simulink model "advanced_active_clamping"  (R2023b)
settings: Solver=ode1be  StartTime=0.0  StopTime=simlength  FixedStep=tc  RelTol=1e-3
values from neighbouring files (symbols this model uses):
  Rgate = 2.5    [init_model.m]
  Rgate_internal = 4    [init_model.m]
  t0_dpt = 5e-6    (= 5e-06)    [init_model.m]
  t1_dpt = t0_dpt + delta_time_first_pulse    (= 0.000105)    [init_model.m]
  t2_dpt = t1_dpt + deadtime    (= 0.000108)    [init_model.m]
  t3_dpt = t2_dpt + delta_time_discharge    (= 0.000128)    [init_model.m]
  t4_dpt = t3_dpt + deadtime    (= 0.000131)    [init_model.m]
  t5_dpt = t4_dpt + delta_time_second_pulse    (= 0.000166)    [init_model.m]
  t6_dpt = t5_dpt + deadtime    (= 0.000169)    [init_model.m]
  Vdc = 1400    [init_model.m]
  Vgate_h = 15    [init_model.m]
  Vgate_l = -7    [init_model.m]
libraries: fl_lib x55, nesl_utility x11, ee_lib x10, simulink x4
(part 1 of 3)
settings Model: SimulationMode=accelerator  Creator=ltnbda  LastModifiedBy=ltnbda

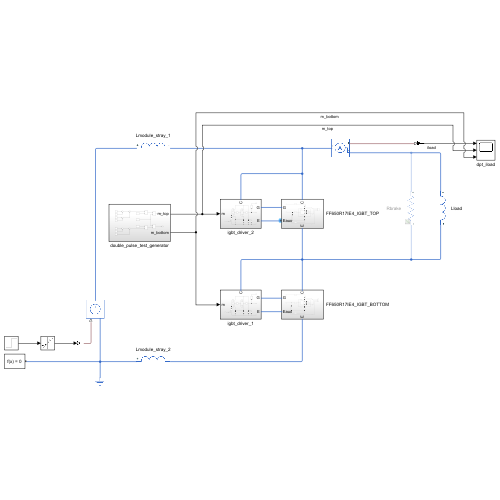
[thumbnail: Simulink's stored preview of the top-level diagram]
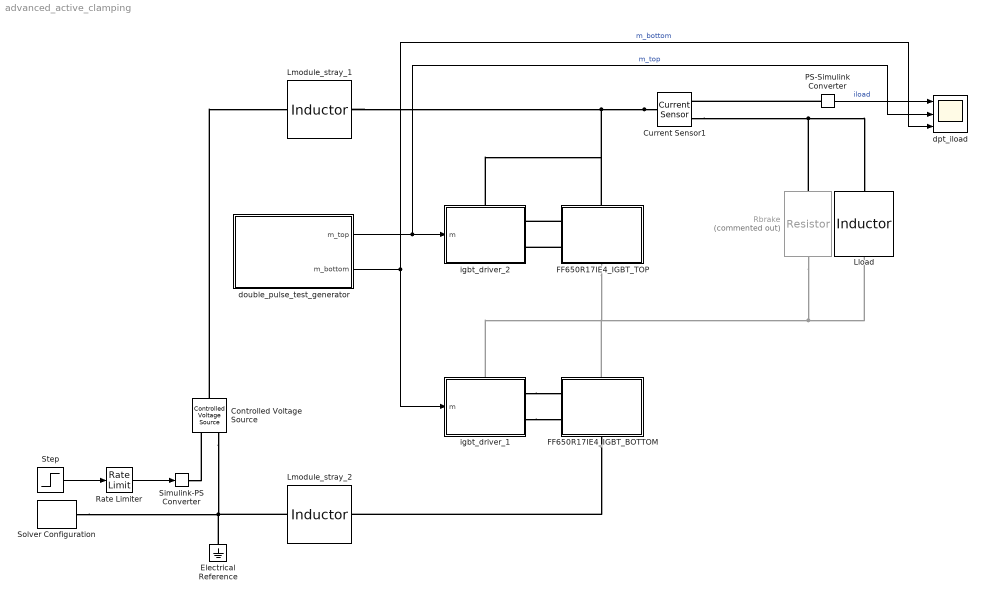
== system advanced_active_clamping ==
  Controlled Voltage Source : fl_lib/Electrical/Electrical Sources/Controlled Voltage Source
  Current Sensor1 : fl_lib/Electrical/Electrical Sensors/Current Sensor
  Electrical Reference : fl_lib/Electrical/Electrical Elements/Electrical Reference
  FF650R17IE4_IGBT_BOTTOM : Subsystem
      settings: PortSchema="{\"entries\":[{\"content\":{\"sides\":[{\"content\":{\"connectorIds\":[\"LConn1\",\"LConn2\"]},\"type\":\"ConnectorPlacement.EquallySpacedRectSide\",\"uuid\":\"ff7886c7-4f8e-447f-95ba-85dce919debf\"},{\"content\":{\"side\":\"RIGHT\"},\"type\":\"ConnectorPlacement.EquallySpacedRectSide\",\"uuid\":\"5b5ddf05-2751-4064-9c00-5bb01a041ae0\"},{\"content\":{\"connectorIds\":[\"LConn3\"],\"side\":\"TOP\"},\"type\":\"ConnectorPlacement.EquallySpacedRectSide\",\"uuid\":\"273e317c-7515-4411-a6b6-783120e9a5d2\"},{\"content\":{\"connectorIds\":[\"RConn1\"],\"side\":\"BOTTOM\"},\"type\":\"ConnectorPlacement.EquallySpacedRectSide\",\"uuid\":\"19a3252d-8455-4daa-8248-ea8f9abc4bb8\"}]},\"type\":\"ConnectorPlacement.EquallySpacedConnector\",\"uuid\":\"2d9de646-1f96-414a-bd08-ff96b52427d0\"}],\"packageUris\":[\"http://schema.mathworks.com/mf0/Connector/R2020b\"],\"version\":\"1.0\"}"
  FF650R17IE4_IGBT_TOP : Subsystem
      settings: PortSchema="{\"entries\":[{\"content\":{\"sides\":[{\"content\":{\"connectorIds\":[\"LConn1\",\"LConn2\"]},\"type\":\"ConnectorPlacement.EquallySpacedRectSide\",\"uuid\":\"ff7886c7-4f8e-447f-95ba-85dce919debf\"},{\"content\":{\"side\":\"RIGHT\"},\"type\":\"ConnectorPlacement.EquallySpacedRectSide\",\"uuid\":\"5b5ddf05-2751-4064-9c00-5bb01a041ae0\"},{\"content\":{\"connectorIds\":[\"LConn3\"],\"side\":\"TOP\"},\"type\":\"ConnectorPlacement.EquallySpacedRectSide\",\"uuid\":\"273e317c-7515-4411-a6b6-783120e9a5d2\"},{\"content\":{\"connectorIds\":[\"RConn1\"],\"side\":\"BOTTOM\"},\"type\":\"ConnectorPlacement.EquallySpacedRectSide\",\"uuid\":\"19a3252d-8455-4daa-8248-ea8f9abc4bb8\"}]},\"type\":\"ConnectorPlacement.EquallySpacedConnector\",\"uuid\":\"2d9de646-1f96-414a-bd08-ff96b52427d0\"}],\"packageUris\":[\"http://schema.mathworks.com/mf0/Connector/R2020b\"],\"version\":\"1.0\"}"
  Lload : fl_lib/Electrical/Electrical Elements/Inductor  l=250e-6 H  r=0 Ohm  g=1e-9 1/Ohm  i_specify=on  i_priority=High  i=0 A  i_nominal_specify=off  i_nominal_unit=A  i_nominal_value=1  v_specify=off  v_priority=None  v=0 V  v_nominal_specify=off  v_nominal_unit=V  v_nominal_value=1  i_L_specify=off  i_L_priority=High  i_L=0 A  i_L_nominal_specify=off  i_L_nominal_unit=A  i_L_nominal_value=1
  Lmodule_stray_1 : fl_lib/Electrical/Electrical Elements/Inductor  l=10e-9 H  r=0 Ohm  g=1e-9 1/Ohm  i_specify=on  i_priority=High  i=0 A  i_nominal_specify=off  i_nominal_unit=A  i_nominal_value=1  v_specify=off  v_priority=None  v=0 V  v_nominal_specify=off  v_nominal_unit=V  v_nominal_value=1  i_L_specify=off  i_L_priority=High  i_L=0 A  i_L_nominal_specify=off  i_L_nominal_unit=A  i_L_nominal_value=1
  Lmodule_stray_2 : fl_lib/Electrical/Electrical Elements/Inductor  l=10e-9 H  r=0 Ohm  g=1e-9 1/Ohm  i_specify=on  i_priority=High  i=0 A  i_nominal_specify=off  i_nominal_unit=A  i_nominal_value=1  v_specify=off  v_priority=None  v=0 V  v_nominal_specify=off  v_nominal_unit=V  v_nominal_value=1  i_L_specify=off  i_L_priority=High  i_L=0 A  i_L_nominal_specify=off  i_L_nominal_unit=A  i_L_nominal_value=1
  PS-Simulink Converter : nesl_utility/PS-Simulink Converter  PhysicalDomain=network_engine_domain  SubClassName=ps_output  LeftPortType=input  RightPortType=output  PseudoPeriodic=off  Frequencies=[]  VectorFormat=1-D array  Unit=A  AffineConversion=off
  Rate Limiter : RateLimiter  RisingSlewLimit=Vdc/t0_dpt  FallingSlewLimit=-Vdc/t0_dpt  SampleTimeMode=inherited
  Rbrake : fl_lib/Electrical/Electrical Elements/Resistor  Commented=on  R=2.5 Ohm  i_specify=off  i_priority=None  i=0 A  i_nominal_specify=off  i_nominal_unit=A  i_nominal_value=1  v_specify=off  v_priority=None  v=0 V  v_nominal_specify=off  v_nominal_unit=V  v_nominal_value=1
  Simulink-PS Converter : nesl_utility/Simulink-PS Converter  PhysicalDomain=network_engine_domain  SubClassName=ps_input  LeftPortType=input  RightPortType=output  PseudoPeriodic=off  Frequencies=[]  NoiseDistribution=none  NoiseParameters=[]  Unit=V  AffineConversion=off  FilteringAndDerivatives=provide  SimscapeFilterOrder=1  InputFilterTimeConstant=0.001  UdotUserProvided=0
  Solver Configuration : nesl_utility/Solver Configuration  PhysicalDomain=network_engine_domain  SubClassName=solver  LeftPortType=input  RightPortType=generic  Tones=[]  Harmonics=[]  SimulateNoise=off  Profile=off  UseLocalSampling=off  EnableSwitchedLinearOptims=on  FrequencyDomain=off  UseCCode=off  RelTol=0.001  AbsTol=0.001  MinStep=1e-09  ToWorkspace=off  RevertToSquareIcSolve=off  NumHomotopyIterations=100  PhasorMode=off  PhasorModeNumHarmonics=1  ConsistencySolver=NEWTON_XTOL_AFTER_FTOL  IndexReductionMethod=DerivativeReplacement  DoDC=off  ResidualTolerance=1e-09  ConsistencyTolSource=GLOBAL  ConsistencyAbsTol=0.001  ConsistencyRelTol=0.001  ConsistencyTolFactor=0.001  UseLocalSolver=on  LocalSolverChoice=NE_BACKWARD_EULER_ADVANCER  ResolveIndetEquations=on  FunctionEvalNumThread=1  LocalSolverSampleTime=tc  DoFixedCost=on  MaxNonlinIter=3  MaxModeIter=2  ComputeImpulses=off  ImpulseIterations=2  LinearAlgebra=auto  LinearAlgebraNumThread=0  EquationFormulation=NE_TIME_EF  DelaysMemoryBudget=1024  AutomaticFiltering=on  FilteringTimeConstant=0.001  PartitionStorageMethod=AS_NEEDED  PartitionMemoryBudget=1024  PartitionMethod=ROBUST  MultibodyUseLocalSolver=off  MultibodyLocalSolverChoice=ODE1  MultibodyLocalSolverSampleTime=0.001
  Step : Step  Time=t0_dpt/2  After=Vdc  SampleTime=0
  double_pulse_test_generator : Subsystem
  dpt_iload : Scope  NumInputPorts=3
  igbt_driver_1 : Subsystem
      settings: PortSchema="{\"entries\":[{\"content\":{\"sides\":[{\"content\":{\"connectorIds\":[\"In1\"]},\"type\":\"ConnectorPlacement.EquallySpacedRectSide\",\"uuid\":\"b5509b55-d3cc-4efd-9891-ed827e6493bc\"},{\"content\":{\"connectorIds\":[\"RConn1\",\"RConn2\"],\"side\":\"RIGHT\"},\"type\":\"ConnectorPlacement.EquallySpacedRectSide\",\"uuid\":\"dc61ae1f-7170-4116-bac1-734370f471cc\"},{\"content\":{\"connectorIds\":[\"LConn1\"],\"side\":\"TOP\"},\"type\":\"ConnectorPlacement.EquallySpacedRectSide\",\"uuid\":\"cf9a77ed-ea6e-4e11-a579-61eb3ec7e471\"},{\"content\":{\"side\":\"BOTTOM\"},\"type\":\"ConnectorPlacement.EquallySpacedRectSide\",\"uuid\":\"ce6ad74e-4413-41a4-ad14-2bad8f537036\"}]},\"type\":\"ConnectorPlacement.EquallySpacedConnector\",\"uuid\":\"97660843-38c1-4e0d-9e7b-61942c4360f8\"}],\"packageUris\":[\"http://schema.mathworks.com/mf0/Connector/R2020b\"],\"version\":\"1.0\"}"
  igbt_driver_2 : Subsystem
      settings: PortSchema="{\"entries\":[{\"content\":{\"sides\":[{\"content\":{\"connectorIds\":[\"In1\"]},\"type\":\"ConnectorPlacement.EquallySpacedRectSide\",\"uuid\":\"b5509b55-d3cc-4efd-9891-ed827e6493bc\"},{\"content\":{\"connectorIds\":[\"RConn1\",\"RConn2\"],\"side\":\"RIGHT\"},\"type\":\"ConnectorPlacement.EquallySpacedRectSide\",\"uuid\":\"dc61ae1f-7170-4116-bac1-734370f471cc\"},{\"content\":{\"connectorIds\":[\"LConn1\"],\"side\":\"TOP\"},\"type\":\"ConnectorPlacement.EquallySpacedRectSide\",\"uuid\":\"cf9a77ed-ea6e-4e11-a579-61eb3ec7e471\"},{\"content\":{\"side\":\"BOTTOM\"},\"type\":\"ConnectorPlacement.EquallySpacedRectSide\",\"uuid\":\"ce6ad74e-4413-41a4-ad14-2bad8f537036\"}]},\"type\":\"ConnectorPlacement.EquallySpacedConnector\",\"uuid\":\"97660843-38c1-4e0d-9e7b-61942c4360f8\"}],\"packageUris\":[\"http://schema.mathworks.com/mf0/Connector/R2020b\"],\"version\":\"1.0\"}"
  wires:
  Step/1 -> Rate Limiter/1
  double_pulse_test_generator/2(m_bottom) -> igbt_driver_1/1(m), dpt_iload/3  "m_bottom"
  double_pulse_test_generator/1(m_top) -> igbt_driver_2/1(m), dpt_iload/2  "m_top"
  PS-Simulink Converter/1 -> dpt_iload/1  "iload"
  Rate Limiter/1 -> Simulink-PS Converter/1
  connections:
  Current Sensor1/LConn1 -- igbt_driver_2/LConn1 -- FF650R17IE4_IGBT_TOP/LConn3 -- Lmodule_stray_1/RConn1
  Simulink-PS Converter/RConn1 -- Controlled Voltage Source/RConn1
  FF650R17IE4_IGBT_BOTTOM/RConn1 -- Lmodule_stray_2/RConn1
  Rbrake/RConn1 -- igbt_driver_1/LConn1 -- FF650R17IE4_IGBT_BOTTOM/LConn3 -- FF650R17IE4_IGBT_TOP/RConn1 -- Lload/RConn1
  igbt_driver_1/RConn1 -- FF650R17IE4_IGBT_BOTTOM/LConn1
  FF650R17IE4_IGBT_TOP/LConn1 -- igbt_driver_2/RConn1
  Current Sensor1/RConn2 -- Rbrake/LConn1 -- Lload/LConn1
  PS-Simulink Converter/LConn1 -- Current Sensor1/RConn1
  Controlled Voltage Source/LConn1 -- Lmodule_stray_1/LConn1
  Lmodule_stray_2/LConn1 -- Electrical Reference/LConn1 -- Controlled Voltage Source/RConn2 -- Solver Configuration/RConn1
  igbt_driver_1/RConn2 -- FF650R17IE4_IGBT_BOTTOM/LConn2
  FF650R17IE4_IGBT_TOP/LConn2 -- igbt_driver_2/RConn2

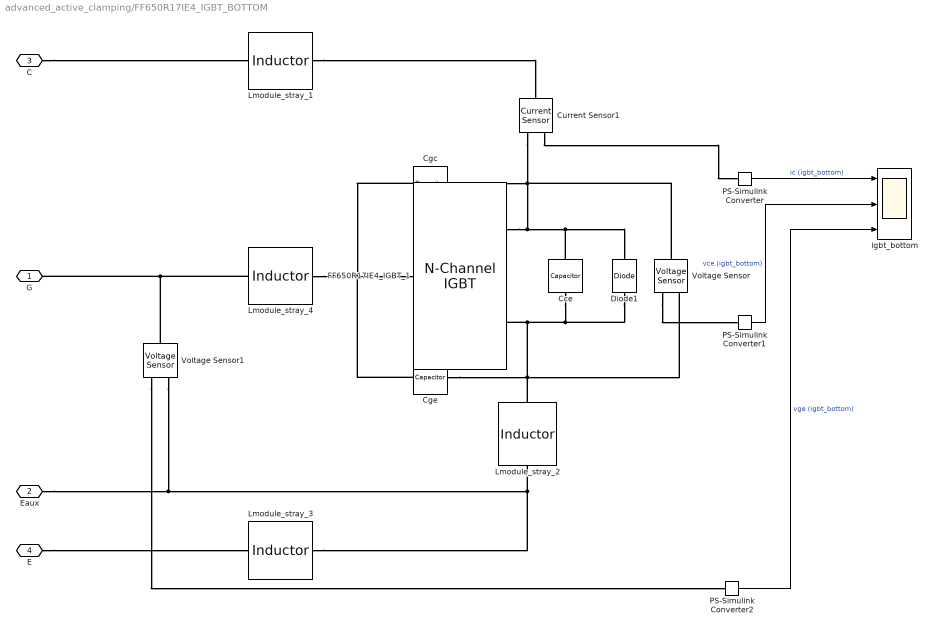
== system advanced_active_clamping/FF650R17IE4_IGBT_BOTTOM ==
  Cce : fl_lib/Electrical/Electrical Elements/Capacitor  c=Cce F  r=RCce Ohm  g=0 1/Ohm  i_specify=off  i_priority=None  i=0 A  i_nominal_specify=off  i_nominal_unit=A  i_nominal_value=1  v_specify=off  v_priority=None  v=0 V  v_nominal_specify=off  v_nominal_unit=V  v_nominal_value=1  vc_specify=off  vc_priority=High  vc=0 V  vc_nominal_specify=off  vc_nominal_unit=V  vc_nominal_value=1
  Cgc : fl_lib/Electrical/Electrical Elements/Capacitor  c=Cgc F  r=RCgc Ohm  g=0 1/Ohm  i_specify=off  i_priority=None  i=0 A  i_nominal_specify=off  i_nominal_unit=A  i_nominal_value=1  v_specify=off  v_priority=None  v=0 V  v_nominal_specify=off  v_nominal_unit=V  v_nominal_value=1  vc_specify=off  vc_priority=High  vc=0 V  vc_nominal_specify=off  vc_nominal_unit=V  vc_nominal_value=1
  Cge : fl_lib/Electrical/Electrical Elements/Capacitor  c=Cge F  r=RCge Ohm  g=0 1/Ohm  i_specify=off  i_priority=None  i=0 A  i_nominal_specify=off  i_nominal_unit=A  i_nominal_value=1  v_specify=off  v_priority=None  v=0 V  v_nominal_specify=off  v_nominal_unit=V  v_nominal_value=1  vc_specify=off  vc_priority=High  vc=0 V  vc_nominal_specify=off  vc_nominal_unit=V  vc_nominal_value=1
  Current Sensor1 : fl_lib/Electrical/Electrical Sensors/Current Sensor
  Diode1 : fl_lib/Electrical/Electrical Elements/Diode  Vf=2 V  Ron=0.3 Ohm  Goff=1e-8 1/Ohm  i_specify=off  i_priority=None  i=0 A  i_nominal_specify=off  i_nominal_unit=A  i_nominal_value=1  v_specify=off  v_priority=None  v=0 V  v_nominal_specify=off  v_nominal_unit=V  v_nominal_value=1
  FF650R17IE4_IGBT_1 : ee_lib/Semiconductors & Converters/N-Channel IGBT  model_type=ee.enum.igbt.parameterization.equation  Ices=5 mA  Vces=1700 V  Vth=5.8 V  Vce_sat=2.35 V  Ice_sat=650 A  Vge_sat=15 V  Tmeas=125 degC  Vge_vec=[-1, 0, 2, 3, 5, 6, 7, 8, 10, 12, 15, 18, 20] V  Vce_vec=[0, .25, .5, .75, 1, 1.26, 1.51, 1.76, 2.01, 2.26, 2.51, 2.76, 3.01, 3.27, 3.52, 3.77, 4.02, 4.27, 4.52, 4.77] V  T_vec=[25, 125] degC  Ic_mat=[0, 0, 0, 0, 0, 0, 0, 0, 0, 0, 0, 0, 0, 0, 0, 0, 0, 0, 0, 0; 0, 0, 0, 0, 0, 0, 0, 0, 0, 0, 0, 0, 0, 0, 0, 0, 0, 0, 0, 0; 0, 0, 0, 0, 0, 0, 0, 0, 0, 0, 0, 0, 0, 0, 0, 0, 0, 0, 0, 0; 0, 0, 0, 0, 0, 0, 0, 0, 0, 0, 0, 0, 0, 0, 0, 0, 0, 0, 0, 0; 0, 0, 0, 0, 0, 0, 0, 0, 0, 0, 0, 0, 0, 0, 0, 0, 0, 0, 0, 0; 0, 0, 0, .81, 3.13, 4.97, 6.03, 6.53, 6.84, 7.01, 7.19, 7.32, 7.44, 7.55, 7.67, 7.78, 7.89, 8, 8.07, 8.07; 0, 0, 0, 1.07, 5.5, 12.93, 22.09, 29.14, 35.27, 38.97, 41.37, 43.08, 44.52, 45.45, 46.28, 46.85, 47.41, 47.76, 48.06, 48.36; 0, 0, 0, 1.1, 6.99, 16.51, 28.38, 41.53, 55.76, 69.08, 80.5, 89.56, 96.13, 101.45, 105.15, 107.99, 110.09, 111.87, 113.54, 114.95; 0, 0, 0, 1.36, 6.26, 17.43, 33.6, 50.43, 71.75, 93.61, 114.64, 134.42, 151.44, 164.25, 177.06, 189.88, 202.69, 215.51, 228.32, 241.14; 0, 0, 0, 1.42, 6.4, 18.7, 36.19, 55.23, 79.71, 106.22, 131.28, 156.62, 182.79, 208.97, 235.15, 261.32, 287.5, 313.67, 339.85, 366.02; 0, 0, 0, 1.45, 6.81, 20.01, 39.61, 60.63, 88.74, 117.7, 147.16, 191.87, 237.14, 282.42, 327.69, 372.96, 418.23, 463.5, 508.77, 554.04; 0, 0, 0, 1.49, 6.97, 20.55, 41.34, 64.15, 94.91, 126.1, 170.16, 233.77, 297.38, 360.98, 424.59, 488.19, 551.8, 615.4, 679.01, 742.62; 0, 0, 0, 1.5, 7.5, 20.96, 42.17, 66.19, 98.34, 131.14, 187.84, 263.46, 339.09, 414.72, 490.34, 565.97, 641.6, 717.22, 792.85, 868.48] A  Ic_mat_3D=zeros(13, 20, 2) A  C_param=ee.enum.igbt.capacitanceParam.fixedciss  C_GE=23.7 nF  C_GC=2.7 nF  C_CE=0 nF  C_ies=54 nF  C_res=1.7 nF  C_oes=0 nF  C_GE_vec=[25, 31, 26.5, 24.9, 25, 24.9, 24.6, 24.7, 24.8] nF  C_GC_vec=[55, 9, 5.5, 3.1, 2.5, 2.1, 1.9, 1.8, 1.7] nF  C_Vge_vec=0 V  C_CE_vec=[5, 11, 6.5, 4.9, 3.5, 2.7, 2.1, 1.7, 1.4] nF  C_ies_vec=[80, 40, 32, 28, 27.5, 27, 26.5, 26.5, 26.5] nF  C_res_vec=[55, 9, 5.5, 3.1, 2.5, 2.1, 1.9, 1.8, 1.7] nF  C_oes_vec=[60, 20, 12, 8, 6, 4.8, 4, 3.5, 3.1] nF  C_Vce_vec=[0, 1, 2, 5, 10, 15, 20, 25, 30] V  charge_linearity_param=ee.enum.igbt.cgcLinearity.constant  C_OX=20 nF  V_C_OX=-5 V  TF=0 us  TT=0 us  ec=1  VAF=1 V  RC=0.001 Ohm  RE=0.001 Ohm  RG=2.3 Ohm  BF=50  T_param=ee.enum.igbt.temperatureParameterization.none  Ices_T2=100 mA  EG=1.11 eV  Vce_sat_T2=3 V  Tmeas2=125 degC  XTI=3  BEX=-1.5  RG_alpha=0 1/K  Tdevice=300 K  Tdevice_3D=25 degC  has_thermal_port=1  ig_specify=off  ig_priority=None  ig=0 A  ig_nominal_specify=off  ig_nominal_unit=A  ig_nominal_value=1  ic_specify=off  ic_priority=None  ic=0 A  ic_nominal_specify=off  ic_nominal_unit=A  ic_nominal_value=1  vge_specify=off  vge_priority=None  vge=0 V  vge_nominal_specify=off  vge_nominal_unit=V  vge_nominal_value=1  vce_specify=off  vce_priority=None  vce=0 V  vce_nominal_specify=off  vce_nominal_unit=V  vce_nominal_value=1  v_Cge_specify=off  v_Cge_priority=High  v_Cge=0 V  v_Cge_nominal_specify=off  v_Cge_nominal_unit=V  v_Cge_nominal_value=1  v_Cce_specify=off  v_Cce_priority=High  v_Cce=0 V  v_Cce_nominal_specify=off  v_Cce_nominal_unit=V  v_Cce_nominal_value=1  thermal_network_parameterization=ee.enum.thermalNetworkTopology.junctionCase  Rth=[0, 10] K/W  Rth_Cauer=[1, 3, 10] K/W  Rth_Foster=[4, 6] K/W  thermal_mass_parameterization=ee.enum.thermalNetwork.timeconstant  thermal_mass=[0, 1] J/K  thermal_mass_Cauer=[.1, .3, 1] J/K  thermal_mass_Foster=[1.5, 3] J/K  thermal_time_constant=[0, 10] s  thermal_time_constant_Cauer=[1, 3, 10] s  thermal_time_constant_Foster=[6, 18] s  thermal_mass_initial_temperatures=[25, 25] degC  thermal_mass_initial_temperatures_Cauer=[25, 25, 25] degC  Tvec_initial_Foster=[25, 25, 25, 25] degC  Ic_vec1=[0, 10, 50, 100, 200, 400, 600] A  Vce_vec1=[0, 1.1, 1.3, 1.45, 1.75, 2.25, 2.7] V  Rmiller=0.1 Ohm  Goff=1e-5 1/Ohm  t_on=0.07 us  t_rise=0.7 us  t_off=0.2 us  t_fall=0.5 us  v_meas=300 V  vStartTurnOn_specify=off  vStartTurnOn_priority=None  vStartTurnOn=1 V  tStartTurnOn_specify=off  tStartTurnOn_priority=None  tStartTurnOn=0 s  vStartTurnOff_specify=off  vStartTurnOff_priority=None  vStartTurnOff=0.5 V  tStartTurnOff_specify=off  tStartTurnOff_priority=None  tStartTurnOff=0 s  Tj_vec1=[298.15, 398.15] K  Vce_mat1=[0, 1.1, 1.3, 1.45, 1.75, 2.25, 2.7; 0, 1, 1.15, 1.35, 1.7, 2.35, 3] V  Tj_vec_loss=[298.15, 398.15] K  Ic_vec_loss=[0, 10, 50, 100, 200, 400, 600] A  E_turn_on_mat1=[0, .2, 1, 2, 4, 8, 15; 0, .3, 1.3, 2.5, 5, 11, 18] * 1e-3 J  E_turn_off_mat1=[0, .3, 1.5, 3, 6, 15, 25; 0, .7, 3.3, 6.5, 13, 25, 35] * 1e-3 J  iStartTurnOff_specify=off  iStartTurnOff_priority=None  iStartTurnOff=0 A  Tdevice_specify=off  Tdevice_priority=None
      settings: InternalSimscapePortConfiguration="{\"Bottom\":[],\"Left\":[{\"id\":\"G\",\"label\":\"\",\"type\":\"foundation.electrical.electrical\"}],\"Right\":[{\"id\":\"C\",\"label\":\"\",\"type\":\"foundation.electrical.electrical\"},{\"id\":\"E\",\"label\":\"\",\"type\":\"foundation.electrical.electrical\"}],\"Top\":[]}"
  Lmodule_stray_{1..4} (4 alike) : fl_lib/Electrical/Electrical Elements/Inductor  l=Lstray_module H  r=RLstray_module Ohm  g=1e-9 1/Ohm  i_specify=on  i_priority=High  i=0 A  i_nominal_specify=off  i_nominal_unit=A  i_nominal_value=1  v_specify=off  v_priority=None  v=0 V  v_nominal_specify=off  v_nominal_unit=V  v_nominal_value=1  i_L_specify=off  i_L_priority=High  i_L=0 A  i_L_nominal_specify=off  i_L_nominal_unit=A  i_L_nominal_value=1
  PS-Simulink Converter : nesl_utility/PS-Simulink Converter  PhysicalDomain=network_engine_domain  SubClassName=ps_output  LeftPortType=input  RightPortType=output  PseudoPeriodic=off  Frequencies=[]  VectorFormat=1-D array  Unit=A  AffineConversion=off
  PS-Simulink Converter1 : nesl_utility/PS-Simulink Converter  PhysicalDomain=network_engine_domain  SubClassName=ps_output  LeftPortType=input  RightPortType=output  PseudoPeriodic=off  Frequencies=[]  VectorFormat=1-D array  Unit=V  AffineConversion=off
  PS-Simulink Converter2 : nesl_utility/PS-Simulink Converter  PhysicalDomain=network_engine_domain  SubClassName=ps_output  LeftPortType=input  RightPortType=output  PseudoPeriodic=off  Frequencies=[]  VectorFormat=1-D array  Unit=V  AffineConversion=off
  Voltage Sensor : fl_lib/Electrical/Electrical Sensors/Voltage Sensor
  Voltage Sensor1 : fl_lib/Electrical/Electrical Sensors/Voltage Sensor
  igbt_bottom : Scope  NumInputPorts=3
  G : PMIOPort  Side=Left
  Eaux : PMIOPort  Port=2  Side=Left
  C : PMIOPort  Port=3  Side=Left
  E : PMIOPort  Port=4  Side=Right
  wires:
  PS-Simulink Converter2/1 -> igbt_bottom/3  "vge (igbt_bottom)"
  PS-Simulink Converter/1 -> igbt_bottom/1  "ic (igbt_bottom)"
  PS-Simulink Converter1/1 -> igbt_bottom/2  "vce (igbt_bottom)"
  connections:
  Lmodule_stray_2/RConn1 -- Voltage Sensor1/RConn2 -- Eaux/RConn1 -- Lmodule_stray_3/LConn1
  G/RConn1 -- Lmodule_stray_4/LConn1 -- Voltage Sensor1/LConn1
  FF650R17IE4_IGBT_1/RConn2 -- Cce/RConn1 -- Diode1/LConn1 -- Lmodule_stray_2/LConn1 -- Voltage Sensor/RConn2 -- Cge/RConn1
  E/RConn1 -- Lmodule_stray_3/RConn1
  C/RConn1 -- Lmodule_stray_1/LConn1
  Lmodule_stray_1/RConn1 -- Current Sensor1/LConn1
  FF650R17IE4_IGBT_1/LConn1 -- Lmodule_stray_4/RConn1 -- Cgc/LConn1 -- Cge/LConn1
  Voltage Sensor1/RConn1 -- PS-Simulink Converter2/LConn1
  Voltage Sensor/RConn1 -- PS-Simulink Converter1/LConn1
  Voltage Sensor/LConn1 -- Current Sensor1/RConn2 -- Cgc/RConn1 -- Diode1/RConn1 -- Cce/LConn1 -- FF650R17IE4_IGBT_1/RConn1
  Current Sensor1/RConn1 -- PS-Simulink Converter/LConn1

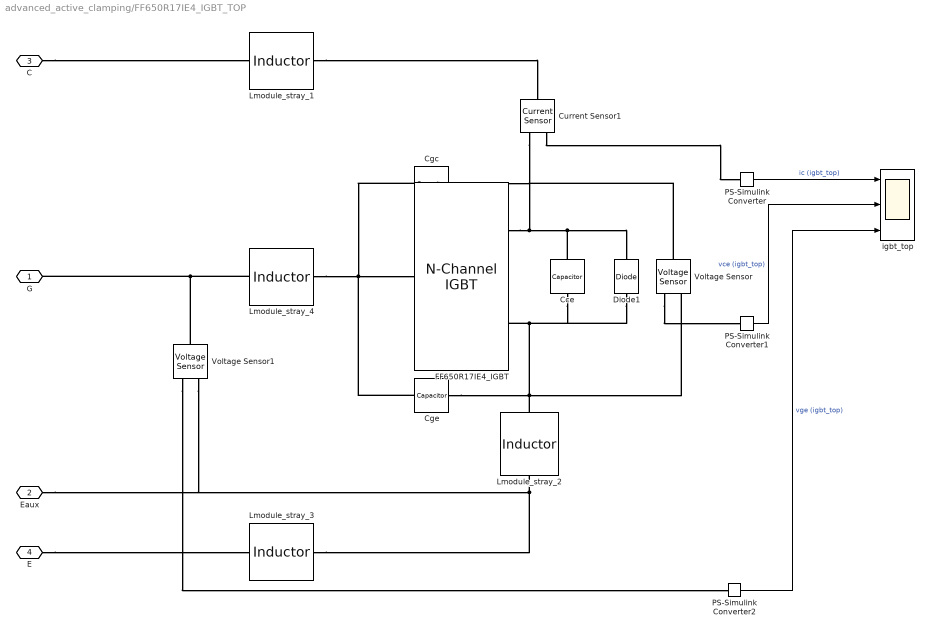
== system advanced_active_clamping/FF650R17IE4_IGBT_TOP ==
  Cce : fl_lib/Electrical/Electrical Elements/Capacitor  c=Cce F  r=RCce Ohm  g=0 1/Ohm  i_specify=off  i_priority=None  i=0 A  i_nominal_specify=off  i_nominal_unit=A  i_nominal_value=1  v_specify=off  v_priority=None  v=0 V  v_nominal_specify=off  v_nominal_unit=V  v_nominal_value=1  vc_specify=off  vc_priority=High  vc=0 V  vc_nominal_specify=off  vc_nominal_unit=V  vc_nominal_value=1
  Cgc : fl_lib/Electrical/Electrical Elements/Capacitor  c=Cgc F  r=RCgc Ohm  g=0 1/Ohm  i_specify=off  i_priority=None  i=0 A  i_nominal_specify=off  i_nominal_unit=A  i_nominal_value=1  v_specify=off  v_priority=None  v=0 V  v_nominal_specify=off  v_nominal_unit=V  v_nominal_value=1  vc_specify=off  vc_priority=High  vc=0 V  vc_nominal_specify=off  vc_nominal_unit=V  vc_nominal_value=1
  Cge : fl_lib/Electrical/Electrical Elements/Capacitor  c=Cge F  r=RCge Ohm  g=0 1/Ohm  i_specify=off  i_priority=None  i=0 A  i_nominal_specify=off  i_nominal_unit=A  i_nominal_value=1  v_specify=off  v_priority=None  v=0 V  v_nominal_specify=off  v_nominal_unit=V  v_nominal_value=1  vc_specify=off  vc_priority=High  vc=0 V  vc_nominal_specify=off  vc_nominal_unit=V  vc_nominal_value=1
  Current Sensor1 : fl_lib/Electrical/Electrical Sensors/Current Sensor
  Diode1 : fl_lib/Electrical/Electrical Elements/Diode  Vf=2 V  Ron=0.3 Ohm  Goff=1e-8 1/Ohm  i_specify=off  i_priority=None  i=0 A  i_nominal_specify=off  i_nominal_unit=A  i_nominal_value=1  v_specify=off  v_priority=None  v=0 V  v_nominal_specify=off  v_nominal_unit=V  v_nominal_value=1
  FF650R17IE4_IGBT : ee_lib/Semiconductors & Converters/N-Channel IGBT  model_type=ee.enum.igbt.parameterization.equation  Ices=5 mA  Vces=1700 V  Vth=5.8 V  Vce_sat=2.35 V  Ice_sat=650 A  Vge_sat=15 V  Tmeas=125 degC  Vge_vec=[-1, 0, 2, 3, 5, 6, 7, 8, 10, 12, 15, 18, 20] V  Vce_vec=[0, .25, .5, .75, 1, 1.26, 1.51, 1.76, 2.01, 2.26, 2.51, 2.76, 3.01, 3.27, 3.52, 3.77, 4.02, 4.27, 4.52, 4.77] V  T_vec=[25, 125] degC  Ic_mat=[0, 0, 0, 0, 0, 0, 0, 0, 0, 0, 0, 0, 0, 0, 0, 0, 0, 0, 0, 0; 0, 0, 0, 0, 0, 0, 0, 0, 0, 0, 0, 0, 0, 0, 0, 0, 0, 0, 0, 0; 0, 0, 0, 0, 0, 0, 0, 0, 0, 0, 0, 0, 0, 0, 0, 0, 0, 0, 0, 0; 0, 0, 0, 0, 0, 0, 0, 0, 0, 0, 0, 0, 0, 0, 0, 0, 0, 0, 0, 0; 0, 0, 0, 0, 0, 0, 0, 0, 0, 0, 0, 0, 0, 0, 0, 0, 0, 0, 0, 0; 0, 0, 0, .81, 3.13, 4.97, 6.03, 6.53, 6.84, 7.01, 7.19, 7.32, 7.44, 7.55, 7.67, 7.78, 7.89, 8, 8.07, 8.07; 0, 0, 0, 1.07, 5.5, 12.93, 22.09, 29.14, 35.27, 38.97, 41.37, 43.08, 44.52, 45.45, 46.28, 46.85, 47.41, 47.76, 48.06, 48.36; 0, 0, 0, 1.1, 6.99, 16.51, 28.38, 41.53, 55.76, 69.08, 80.5, 89.56, 96.13, 101.45, 105.15, 107.99, 110.09, 111.87, 113.54, 114.95; 0, 0, 0, 1.36, 6.26, 17.43, 33.6, 50.43, 71.75, 93.61, 114.64, 134.42, 151.44, 164.25, 177.06, 189.88, 202.69, 215.51, 228.32, 241.14; 0, 0, 0, 1.42, 6.4, 18.7, 36.19, 55.23, 79.71, 106.22, 131.28, 156.62, 182.79, 208.97, 235.15, 261.32, 287.5, 313.67, 339.85, 366.02; 0, 0, 0, 1.45, 6.81, 20.01, 39.61, 60.63, 88.74, 117.7, 147.16, 191.87, 237.14, 282.42, 327.69, 372.96, 418.23, 463.5, 508.77, 554.04; 0, 0, 0, 1.49, 6.97, 20.55, 41.34, 64.15, 94.91, 126.1, 170.16, 233.77, 297.38, 360.98, 424.59, 488.19, 551.8, 615.4, 679.01, 742.62; 0, 0, 0, 1.5, 7.5, 20.96, 42.17, 66.19, 98.34, 131.14, 187.84, 263.46, 339.09, 414.72, 490.34, 565.97, 641.6, 717.22, 792.85, 868.48] A  Ic_mat_3D=zeros(13, 20, 2) A  C_param=ee.enum.igbt.capacitanceParam.fixedciss  C_GE=23.7 nF  C_GC=2.7 nF  C_CE=0 nF  C_ies=54 nF  C_res=1.7 nF  C_oes=0 nF  C_GE_vec=[25, 31, 26.5, 24.9, 25, 24.9, 24.6, 24.7, 24.8] nF  C_GC_vec=[55, 9, 5.5, 3.1, 2.5, 2.1, 1.9, 1.8, 1.7] nF  C_Vge_vec=0 V  C_CE_vec=[5, 11, 6.5, 4.9, 3.5, 2.7, 2.1, 1.7, 1.4] nF  C_ies_vec=[80, 40, 32, 28, 27.5, 27, 26.5, 26.5, 26.5] nF  C_res_vec=[55, 9, 5.5, 3.1, 2.5, 2.1, 1.9, 1.8, 1.7] nF  C_oes_vec=[60, 20, 12, 8, 6, 4.8, 4, 3.5, 3.1] nF  C_Vce_vec=[0, 1, 2, 5, 10, 15, 20, 25, 30] V  charge_linearity_param=ee.enum.igbt.cgcLinearity.constant  C_OX=20 nF  V_C_OX=-5 V  TF=0 us  TT=0 us  ec=1  VAF=1 V  RC=0.001 Ohm  RE=0.001 Ohm  RG=2.3 Ohm  BF=50  T_param=ee.enum.igbt.temperatureParameterization.none  Ices_T2=100 mA  EG=1.11 eV  Vce_sat_T2=3 V  Tmeas2=125 degC  XTI=3  BEX=-1.5  RG_alpha=0 1/K  Tdevice=300 K  Tdevice_3D=25 degC  has_thermal_port=1  ig_specify=off  ig_priority=None  ig=0 A  ig_nominal_specify=off  ig_nominal_unit=A  ig_nominal_value=1  ic_specify=off  ic_priority=None  ic=0 A  ic_nominal_specify=off  ic_nominal_unit=A  ic_nominal_value=1  vge_specify=off  vge_priority=None  vge=0 V  vge_nominal_specify=off  vge_nominal_unit=V  vge_nominal_value=1  vce_specify=off  vce_priority=None  vce=0 V  vce_nominal_specify=off  vce_nominal_unit=V  vce_nominal_value=1  v_Cge_specify=off  v_Cge_priority=High  v_Cge=0 V  v_Cge_nominal_specify=off  v_Cge_nominal_unit=V  v_Cge_nominal_value=1  v_Cce_specify=off  v_Cce_priority=High  v_Cce=0 V  v_Cce_nominal_specify=off  v_Cce_nominal_unit=V  v_Cce_nominal_value=1  thermal_network_parameterization=ee.enum.thermalNetworkTopology.junctionCase  Rth=[0, 10] K/W  Rth_Cauer=[1, 3, 10] K/W  Rth_Foster=[4, 6] K/W  thermal_mass_parameterization=ee.enum.thermalNetwork.timeconstant  thermal_mass=[0, 1] J/K  thermal_mass_Cauer=[.1, .3, 1] J/K  thermal_mass_Foster=[1.5, 3] J/K  thermal_time_constant=[0, 10] s  thermal_time_constant_Cauer=[1, 3, 10] s  thermal_time_constant_Foster=[6, 18] s  thermal_mass_initial_temperatures=[25, 25] degC  thermal_mass_initial_temperatures_Cauer=[25, 25, 25] degC  Tvec_initial_Foster=[25, 25, 25, 25] degC  Ic_vec1=[0, 10, 50, 100, 200, 400, 600] A  Vce_vec1=[0, 1.1, 1.3, 1.45, 1.75, 2.25, 2.7] V  Rmiller=0.1 Ohm  Goff=1e-5 1/Ohm  t_on=0.07 us  t_rise=0.7 us  t_off=0.2 us  t_fall=0.5 us  v_meas=300 V  vStartTurnOn_specify=off  vStartTurnOn_priority=None  vStartTurnOn=1 V  tStartTurnOn_specify=off  tStartTurnOn_priority=None  tStartTurnOn=0 s  vStartTurnOff_specify=off  vStartTurnOff_priority=None  vStartTurnOff=0.5 V  tStartTurnOff_specify=off  tStartTurnOff_priority=None  tStartTurnOff=0 s  Tj_vec1=[298.15, 398.15] K  Vce_mat1=[0, 1.1, 1.3, 1.45, 1.75, 2.25, 2.7; 0, 1, 1.15, 1.35, 1.7, 2.35, 3] V  Tj_vec_loss=[298.15, 398.15] K  Ic_vec_loss=[0, 10, 50, 100, 200, 400, 600] A  E_turn_on_mat1=[0, .2, 1, 2, 4, 8, 15; 0, .3, 1.3, 2.5, 5, 11, 18] * 1e-3 J  E_turn_off_mat1=[0, .3, 1.5, 3, 6, 15, 25; 0, .7, 3.3, 6.5, 13, 25, 35] * 1e-3 J  iStartTurnOff_specify=off  iStartTurnOff_priority=None  iStartTurnOff=0 A  Tdevice_specify=off  Tdevice_priority=None
      settings: InternalSimscapePortConfiguration="{\"Bottom\":[],\"Left\":[{\"id\":\"G\",\"label\":\"\",\"type\":\"foundation.electrical.electrical\"}],\"Right\":[{\"id\":\"C\",\"label\":\"\",\"type\":\"foundation.electrical.electrical\"},{\"id\":\"E\",\"label\":\"\",\"type\":\"foundation.electrical.electrical\"}],\"Top\":[]}"
  Lmodule_stray_{1..4} (4 alike) : fl_lib/Electrical/Electrical Elements/Inductor  l=Lstray_module H  r=RLstray_module Ohm  g=1e-9 1/Ohm  i_specify=on  i_priority=High  i=0 A  i_nominal_specify=off  i_nominal_unit=A  i_nominal_value=1  v_specify=off  v_priority=None  v=0 V  v_nominal_specify=off  v_nominal_unit=V  v_nominal_value=1  i_L_specify=off  i_L_priority=High  i_L=0 A  i_L_nominal_specify=off  i_L_nominal_unit=A  i_L_nominal_value=1
  PS-Simulink Converter : nesl_utility/PS-Simulink Converter  PhysicalDomain=network_engine_domain  SubClassName=ps_output  LeftPortType=input  RightPortType=output  PseudoPeriodic=off  Frequencies=[]  VectorFormat=1-D array  Unit=A  AffineConversion=off
  PS-Simulink Converter1 : nesl_utility/PS-Simulink Converter  PhysicalDomain=network_engine_domain  SubClassName=ps_output  LeftPortType=input  RightPortType=output  PseudoPeriodic=off  Frequencies=[]  VectorFormat=1-D array  Unit=V  AffineConversion=off
  PS-Simulink Converter2 : nesl_utility/PS-Simulink Converter  PhysicalDomain=network_engine_domain  SubClassName=ps_output  LeftPortType=input  RightPortType=output  PseudoPeriodic=off  Frequencies=[]  VectorFormat=1-D array  Unit=V  AffineConversion=off
  Voltage Sensor : fl_lib/Electrical/Electrical Sensors/Voltage Sensor
  Voltage Sensor1 : fl_lib/Electrical/Electrical Sensors/Voltage Sensor
  igbt_top : Scope  NumInputPorts=3
  G : PMIOPort  Side=Left
  Eaux : PMIOPort  Port=2  Side=Left
  C : PMIOPort  Port=3  Side=Left
  E : PMIOPort  Port=4  Side=Right
  wires:
  PS-Simulink Converter1/1 -> igbt_top/2  "vce (igbt_top)"
  PS-Simulink Converter/1 -> igbt_top/1  "ic (igbt_top)"
  PS-Simulink Converter2/1 -> igbt_top/3  "vge (igbt_top)"
  connections:
  Current Sensor1/RConn1 -- PS-Simulink Converter/LConn1
  FF650R17IE4_IGBT/RConn1 -- Cce/LConn1 -- Diode1/RConn1 -- Cgc/RConn1 -- Current Sensor1/RConn2 -- Voltage Sensor/LConn1
  Voltage Sensor/RConn1 -- PS-Simulink Converter1/LConn1
  Voltage Sensor1/RConn1 -- PS-Simulink Converter2/LConn1
  Lmodule_stray_4/RConn1 -- Cge/LConn1 -- FF650R17IE4_IGBT/LConn1 -- Cgc/LConn1
  Lmodule_stray_1/RConn1 -- Current Sensor1/LConn1
  C/RConn1 -- Lmodule_stray_1/LConn1
  E/RConn1 -- Lmodule_stray_3/RConn1
  Lmodule_stray_2/LConn1 -- Voltage Sensor/RConn2 -- Cge/RConn1 -- Diode1/LConn1 -- Cce/RConn1 -- FF650R17IE4_IGBT/RConn2
  Lmodule_stray_4/LConn1 -- Voltage Sensor1/LConn1 -- G/RConn1
  Lmodule_stray_3/LConn1 -- Eaux/RConn1 -- Voltage Sensor1/RConn2 -- Lmodule_stray_2/RConn1

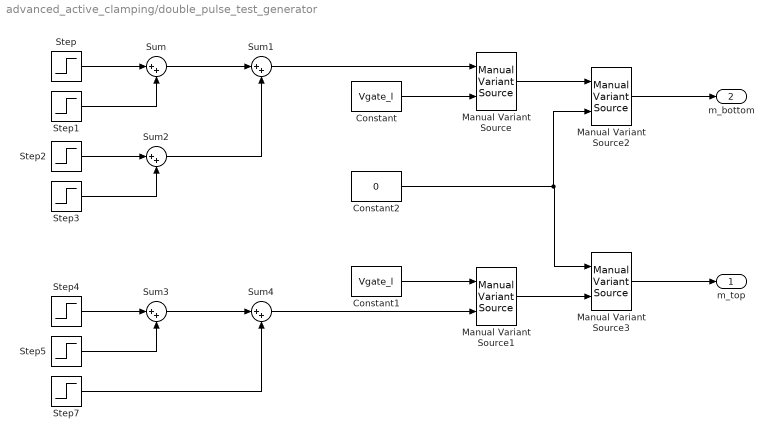
== system advanced_active_clamping/double_pulse_test_generator ==
  Constant : Constant  Value=Vgate_l
  Constant1 : Constant  Value=Vgate_l
  Constant2 : Constant  Value=0
  Manual Variant Source : simulink/Signal Routing/Manual Variant Source  NumChoices=2  LabelModeActiveChoice=V_1
  Manual Variant Source1 : simulink/Signal Routing/Manual Variant Source  NumChoices=2  LabelModeActiveChoice=V_2
  Manual Variant Source2 : simulink/Signal Routing/Manual Variant Source  NumChoices=2  LabelModeActiveChoice=V_1
  Manual Variant Source3 : simulink/Signal Routing/Manual Variant Source  NumChoices=2  LabelModeActiveChoice=V_2
  Step : Step  Time=t0_dpt  Before=Vgate_l  After=Vgate_h  SampleTime=0
  Step1 : Step  Time=t1_dpt  After=-Vgate_h+Vgate_l  SampleTime=0
  Step2 : Step  Time=t4_dpt  After=Vgate_h-Vgate_l  SampleTime=0
  Step3 : Step  Time=t5_dpt  After=-Vgate_h+Vgate_l  SampleTime=0
  Step4 : Step  Time=t2_dpt  Before=Vgate_l  After=Vgate_h  SampleTime=0
  Step5 : Step  Time=t3_dpt  After=-Vgate_h+Vgate_l  SampleTime=0
  Step7 : Step  Time=t6_dpt  After=Vgate_h-Vgate_l  SampleTime=0
  Sum{,1..4} (5 alike) : Sum  Inputs=|++
  m_top : Outport
  m_bottom : Outport  Port=2
  wires:
  Sum/1 -> Sum1/1
  Step/1 -> Sum/1
  Step4/1 -> Sum3/1
  Sum2/1 -> Sum1/2
  Step5/1 -> Sum3/2
  Step1/1 -> Sum/2
  Step2/1 -> Sum2/1
  Step3/1 -> Sum2/2
  Sum3/1 -> Sum4/1
  Step7/1 -> Sum4/2
  Sum1/1 -> Manual Variant Source/1
  Constant/1 -> Manual Variant Source/2
  Manual Variant Source/1 -> Manual Variant Source2/1
  Manual Variant Source2/1 -> m_bottom/1
  Manual Variant Source1/1 -> Manual Variant Source3/2
  Constant1/1 -> Manual Variant Source1/1
  Sum4/1 -> Manual Variant Source1/2
  Constant2/1 -> Manual Variant Source2/2, Manual Variant Source3/1
  Manual Variant Source3/1 -> m_top/1
